simulink model "pumacherif"  (R2023b)
settings: Solver=VariableStepAuto  StartTime=0.0  StopTime=10.0  RelTol=1e-3  AbsTol=1e-3  EnableMultiTasking=on
undefined symbols (not defined in the file): X, Y, Z
libraries: sm_lib x29, nesl_utility x10
settings Model: Creator=echerif913  LastModifiedBy=enzoc
settings SolverCC: AutoScaleAbsTol=off  AlgebraicLoopSolver=TrustRegion  MaxZcPerStep=1
settings DataIOCC: LimitDataPoints=on  MaxDataPoints=10000
settings OptimizationCC: ReuseModelBlockBuffer=off  LifeSpan=inf
settings DebuggingCC: UnconnectedInputMsg=warning  UnconnectedOutputMsg=warning  UnconnectedLineMsg=warning  AllowSymbolicDim=off  SFUnexpectedBacktrackingDiag=warning  SFNoUnconditionalDefaultTransitionDiag=warning  SFExecutionAtInitializationDiag=none  ArithmeticOperatorsInVariantConditions=warning
settings ModelReferenceCC: EnableRefExpFcnMdlSchedulingChecks=on
settings SFSimCC: SimUseLocalCustomCode=off  CustomCodeUndefinedFunction=UseInterfaceOnly
settings RTWCC: RTWUseLocalCustomCode=off  DLArmComputeVersion=19.05
settings CodeAppCC: StateflowObjectComments=on
settings GRTTargetCC: TargetLangStandard=C89/C90 (ANSI)
settings ConfigComp: CovMetricSettings=dw  CovSaveCumulativeToWorkspaceVar=on  CovSaveSingleToWorkspaceVar=on  CovExternalEMLEnable=off  CovSFcnEnable=off
settings SimscapeCC: SimscapeLogType=all  SimscapeLogSimulationStatistics=on  SimscapeLogDataHistory=10000

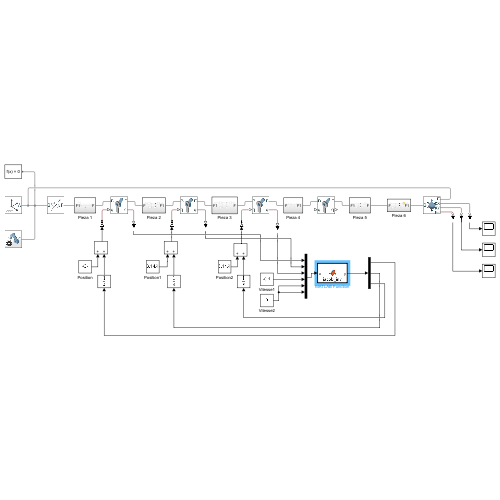
[thumbnail: Simulink's stored preview of the top-level diagram]
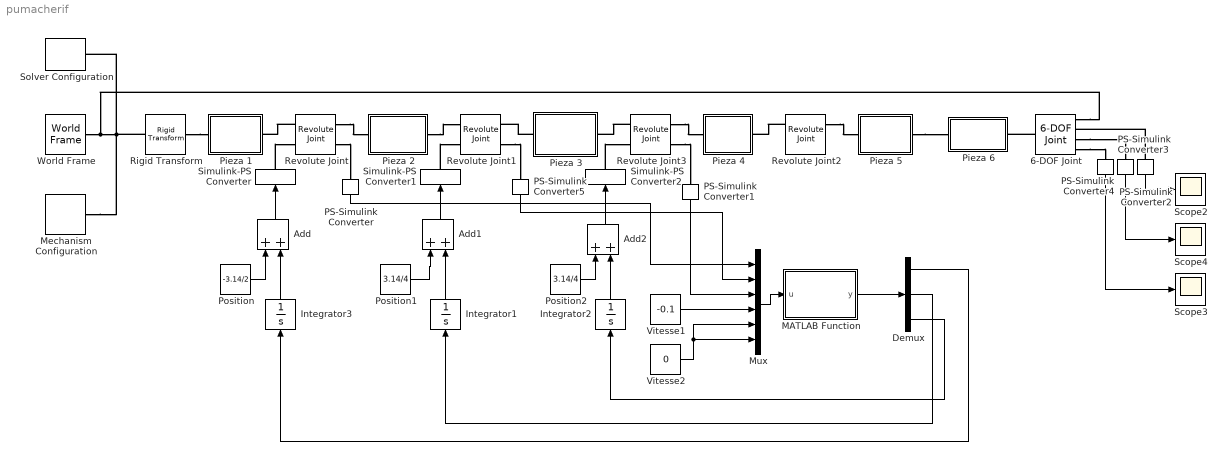
== system pumacherif ==
  6-DOF Joint : sm_lib/Joints/6-DOF Joint  JointMode=Normal  SenseConstraintForce=off  SenseConstraintForceX=off  SenseConstraintForceY=off  SenseConstraintForceZ=off  SenseConstraintTorque=off  SenseConstraintTorqueX=off  SenseConstraintTorqueY=off  SenseConstraintTorqueZ=off  SenseTotalForce=off  SenseTotalForceX=off  SenseTotalForceY=off  SenseTotalForceZ=off  SenseTotalTorque=off  SenseTotalTorqueX=off  SenseTotalTorqueY=off  SenseTotalTorqueZ=off  CompositeWrenchDir=FollowerOnBase  CompositeWrenchFrame=BaseFrame  PxEquilibriumPosition=0  PxEquilibriumPositionUnits=m  PxSpringStiffness=0  PxSpringStiffnessUnits=N/m  PxDampingCoefficient=0  PxDampingCoefficientUnits=N/(m/s)  PxTorqueActuationMode=NoTorque  PxMotionActuationMode=ComputedMotion  PxSensePosition=on  PxSenseVelocity=off  PxSenseAcceleration=off  PxSenseTorqueForce=off  PxSenseLowerLimitTorqueForce=off  PxSenseUpperLimitTorqueForce=off  PxLowerLimitSpecify=off  PxLowerLimitBound=-1  PxLowerLimitBoundUnits=m  PxLowerLimitStiffness=1e6  PxLowerLimitStiffnessUnits=N/m  PxLowerLimitDamping=1e3  PxLowerLimitDampingUnits=N/(m/s)  PxLowerLimitTransitionRegionWidth=1e-4  PxLowerLimitTransitionRegionWidthUnits=m  PxUpperLimitSpecify=off  PxUpperLimitBound=1  PxUpperLimitBoundUnits=m  PxUpperLimitStiffness=1e6  PxUpperLimitStiffnessUnits=N/m  PxUpperLimitDamping=1e3  PxUpperLimitDampingUnits=N/(m/s)  PxUpperLimitTransitionRegionWidth=1e-4  PxUpperLimitTransitionRegionWidthUnits=m  PxPositionTargetSpecify=off  PxPositionTargetPriority=High  PxPositionTargetValue=0  PxPositionTargetValueUnits=m  PxVelocityTargetSpecify=off  PxVelocityTargetPriority=High  PxVelocityTargetValue=0  PxVelocityTargetValueUnits=m/s  PyEquilibriumPosition=0  PyEquilibriumPositionUnits=m  PySpringStiffness=0  PySpringStiffnessUnits=N/m  PyDampingCoefficient=0  PyDampingCoefficientUnits=N/(m/s)  PyTorqueActuationMode=NoTorque  PyMotionActuationMode=ComputedMotion  PySensePosition=on  PySenseVelocity=off  PySenseAcceleration=off  PySenseTorqueForce=off  PySenseLowerLimitTorqueForce=off  PySenseUpperLimitTorqueForce=off  PyLowerLimitSpecify=off  PyLowerLimitBound=-1  PyLowerLimitBoundUnits=m  PyLowerLimitStiffness=1e6  PyLowerLimitStiffnessUnits=N/m  PyLowerLimitDamping=1e3  PyLowerLimitDampingUnits=N/(m/s)  PyLowerLimitTransitionRegionWidth=1e-4  PyLowerLimitTransitionRegionWidthUnits=m  PyUpperLimitSpecify=off  PyUpperLimitBound=1  PyUpperLimitBoundUnits=m  PyUpperLimitStiffness=1e6  PyUpperLimitStiffnessUnits=N/m  PyUpperLimitDamping=1e3  PyUpperLimitDampingUnits=N/(m/s)  PyUpperLimitTransitionRegionWidth=1e-4  PyUpperLimitTransitionRegionWidthUnits=m  PyPositionTargetSpecify=off  PyPositionTargetPriority=High  PyPositionTargetValue=0  PyPositionTargetValueUnits=m  PyVelocityTargetSpecify=off  PyVelocityTargetPriority=High  PyVelocityTargetValue=0  PyVelocityTargetValueUnits=m/s  PzEquilibriumPosition=0  PzEquilibriumPositionUnits=m  PzSpringStiffness=0  PzSpringStiffnessUnits=N/m  PzDampingCoefficient=0  PzDampingCoefficientUnits=N/(m/s)  PzTorqueActuationMode=NoTorque  PzMotionActuationMode=ComputedMotion  PzSensePosition=on  PzSenseVelocity=off  PzSenseAcceleration=off  PzSenseTorqueForce=off  PzSenseLowerLimitTorqueForce=off  PzSenseUpperLimitTorqueForce=off  PzLowerLimitSpecify=off  PzLowerLimitBound=-1  PzLowerLimitBoundUnits=m  PzLowerLimitStiffness=1e6  PzLowerLimitStiffnessUnits=N/m  PzLowerLimitDamping=1e3  PzLowerLimitDampingUnits=N/(m/s)  PzLowerLimitTransitionRegionWidth=1e-4  PzLowerLimitTransitionRegionWidthUnits=m  PzUpperLimitSpecify=off  PzUpperLimitBound=1  PzUpperLimitBoundUnits=m  PzUpperLimitStiffness=1e6  PzUpperLimitStiffnessUnits=N/m  PzUpperLimitDamping=1e3  PzUpperLimitDampingUnits=N/(m/s)  PzUpperLimitTransitionRegionWidth=1e-4  PzUpperLimitTransitionRegionWidthUnits=m  PzPositionTargetSpecify=off  PzPositionTargetPriority=High  PzPositionTargetValue=0  PzPositionTargetValueUnits=m  PzVelocityTargetSpecify=off  PzVelocityTargetPriority=High  PzVelocityTargetValue=0  PzVelocityTargetValueUnits=m/s  SphEqPosRotationMethod=None  SphEqPosRotationAngleUnits=deg  SphEqPosRotationStandardAxis=+Z  SphEqPosRotationAngle=0.0  SphEqPosRotationArbitraryAxis=[0 0 1]  SphEqPosFollAlignAxisA=+X  SphEqPosBaseAlignAxisA=+Y  SphEqPosFollAlignAxisB=+Y  SphEqPosBaseAlignAxisB=+Z  SphEqPosRotationSequenceAxes=FollowerAxes  SphEqPosRotationSequence=XYX  SphEqPosRotationSequenceAngles=[0 0 0]  SphEqPosRotationSequenceAnglesUnits=deg  SphEqPosRotationMatrix=[1 0 0; 0 1 0; 0 0 1]  SphEqPosQuaternion=[1 0 0 0]  SphSpringStiffness=0  SphSpringStiffnessUnits=N*m/deg  SphDampingCoefficient=0  SphDampingCoefficientUnits=N*m/(deg/s)  SphActuateTorqueX=off  SphActuateTorqueY=off  SphActuateTorqueZ=off  SphActuateTorque=off  SphTorqueActuationMode=NoTorque  SphMotionActuationMode=ComputedMotion  SphActuationFrame=BaseFrame  SphSensePosition=off  SphSenseVelocityX=off  SphSenseVelocityY=off  SphSenseVelocityZ=off  SphSenseVelocity=off  SphSenseAccelerationX=off  SphSenseAccelerationY=off  SphSenseAccelerationZ=off  SphSenseAcceleration=off  SphSenseTorqueX=off  SphSenseTorqueY=off  SphSenseTorqueZ=off  SphSenseTorqueForce=off  SphSenseLowerLimitTorqueMag=off  SphSenseUpperLimitTorqueMag=off  SphSensingFrame=BaseFrame  SphLowerLimitSpecify=off  SphLowerLimitBound=15  SphLowerLimitBoundUnits=deg  SphLowerLimitStiffness=1e4  SphLowerLimitStiffnessUnits=N*m/deg  SphLowerLimitDamping=10  SphLowerLimitDampingUnits=N*m/(deg/s)  SphLowerLimitTransitionRegionWidth=0.1  SphLowerLimitTransitionRegionWidthUnits=deg  SphUpperLimitSpecify=off  SphUpperLimitBound=45  SphUpperLimitBoundUnits=deg  SphUpperLimitStiffness=1e4  SphUpperLimitStiffnessUnits=N*m/deg  SphUpperLimitDamping=10  SphUpperLimitDampingUnits=N*m/(deg/s)  SphUpperLimitTransitionRegionWidth=0.1  SphUpperLimitTransitionRegionWidthUnits=deg  SphPositionTargetRotationMethod=None  SphPositionTargetRotationAngleUnits=deg  SphPositionTargetRotationStandardAxis=+Z  SphPositionTargetRotationAngle=0.0  SphPositionTargetRotationArbitraryAxis=[0 0 1]  SphPositionTargetFollAlignAxisA=+X  SphPositionTargetBaseAlignAxisA=+Y  SphPositionTargetFollAlignAxisB=+Y  SphPositionTargetBaseAlignAxisB=+Z  SphPositionTargetRotationSequenceAxes=FollowerAxes  SphPositionTargetRotationSequence=XYX  SphPositionTargetRotationSequenceAngles=[0 0 0]  SphPositionTargetRotationSequenceAnglesUnits=deg  SphPositionTargetRotationMatrix=[1 0 0; 0 1 0; 0 0 1]  SphPositionTargetQuaternion=[1 0 0 0]  SphPositionTargetSpecify=off  SphPositionTargetPriority=High  SphVelocityTargetValue=[0 0 0]  SphVelocityTargetValueUnits=deg/s  SphVelocityTargetSpecify=off  SphVelocityTargetPriority=High  SphVelocityTargetInFollowerFrame=on
  Add : Sum
  Add1 : Sum
  Add2 : Sum
  Demux : Demux  Outputs=3
  Integrator1 : Integrator
  Integrator2 : Integrator
  Integrator3 : Integrator
  MATLAB Function : MATLAB Function  TreatAsAtomicUnit=on
  Mechanism Configuration : sm_lib/Utilities/Mechanism Configuration  UniformGravity=Constant  GravityVector=[0 0 -9.80665]  GravityVectorUnits=m/s^2  LinearizationDelta=0.001  JointModeTransitionNonlinearIterations=2
  Mux : Mux  Inputs=6
  PS-Simulink Converter{,1..5} (6 alike) : nesl_utility/PS-Simulink Converter  PhysicalDomain=network_engine_domain  SubClassName=ps_output  LeftPortType=input  RightPortType=output  PseudoPeriodic=off  Frequencies=[]  VectorFormat=inherit  Unit=inherit  AffineConversion=off
  Pieza 1 : Subsystem
  Pieza 2 : Subsystem
  Pieza 3 : Subsystem
  Pieza 4 : Subsystem
  Pieza 5 : Subsystem
  Pieza 6 : Subsystem
  Position : Constant  Value=-3.14/2
  Position1 : Constant  Value=3.14/4
  Position2 : Constant  Value=3.14/4
  Revolute Joint{,1..3} (4 alike) : sm_lib/Joints/Revolute Joint  JointMode=Normal  SenseConstraintForce=off  SenseConstraintForceX=off  SenseConstraintForceY=off  SenseConstraintForceZ=off  SenseConstraintTorque=off  SenseConstraintTorqueX=off  SenseConstraintTorqueY=off  SenseConstraintTorqueZ=off  SenseTotalForce=off  SenseTotalForceX=off  SenseTotalForceY=off  SenseTotalForceZ=off  SenseTotalTorque=off  SenseTotalTorqueX=off  SenseTotalTorqueY=off  SenseTotalTorqueZ=off  CompositeWrenchDir=FollowerOnBase  CompositeWrenchFrame=BaseFrame  EquilibriumPosition=0  EquilibriumPositionUnits=deg  SpringStiffness=0  SpringStiffnessUnits=N*m/deg  DampingCoefficient=0  DampingCoefficientUnits=N*m/(deg/s)  TorqueActuationMode=ComputedTorque  MotionActuationMode=InputMotion  SensePosition=on  SenseVelocity=off  SenseAcceleration=off  SenseTorqueForce=off  SenseLowerLimitTorqueForce=off  SenseUpperLimitTorqueForce=off  LowerLimitSpecify=off  LowerLimitBound=-90  LowerLimitBoundUnits=deg  LowerLimitStiffness=1e4  LowerLimitStiffnessUnits=N*m/deg  LowerLimitDamping=10  LowerLimitDampingUnits=N*m/(deg/s)  LowerLimitTransitionRegionWidth=0.1  LowerLimitTransitionRegionWidthUnits=deg  UpperLimitSpecify=off  UpperLimitBound=90  UpperLimitBoundUnits=deg  UpperLimitStiffness=1e4  UpperLimitStiffnessUnits=N*m/deg  UpperLimitDamping=10  UpperLimitDampingUnits=N*m/(deg/s)  UpperLimitTransitionRegionWidth=0.1  UpperLimitTransitionRegionWidthUnits=deg  PositionTargetSpecify=off  PositionTargetPriority=High  PositionTargetValue=0  PositionTargetValueUnits=deg  VelocityTargetSpecify=off  VelocityTargetPriority=High  VelocityTargetValue=0  VelocityTargetValueUnits=deg/s
  Rigid Transform : sm_lib/Frames and Transforms/Rigid Transform  TranslationMethod=None  TranslationStandardOffset=0  TranslationStandardOffsetUnits=m  TranslationStandardAxis=+Z  TranslationCartesianOffset=[0 0 0]  TranslationCartesianOffsetUnits=m  TranslationROffset=0  TranslationROffsetUnits=m  TranslationZOffset=0  TranslationZOffsetUnits=m  TranslationThetaOffset=0  TranslationThetaOffsetUnits=deg  RotationMethod=RotationMatrix  RotationAngleUnits=deg  RotationStandardAxis=+Z  RotationAngle=0.0  RotationArbitraryAxis=[0 0 1]  FollAlignAxisA=+X  BaseAlignAxisA=+Y  FollAlignAxisB=+Y  BaseAlignAxisB=+Z  RotationSequenceAxes=FollowerAxes  RotationSequence=XYX  RotationSequenceAngles=[0 0 0]  RotationSequenceAnglesUnits=deg  RotationMatrix=[0 0 1; 1 0 0; 0 1 0]  Quaternion=[1 0 0 0]
  Scope2 : Scope
  Scope3 : Scope
  Scope4 : Scope
  Simulink-PS Converter : nesl_utility/Simulink-PS Converter  PhysicalDomain=network_engine_domain  SubClassName=ps_input  LeftPortType=input  RightPortType=output  PseudoPeriodic=off  Frequencies=[]  NoiseDistribution=none  NoiseParameters=[]  Unit=rad  AffineConversion=off  FilteringAndDerivatives=filter  SimscapeFilterOrder=2  InputFilterTimeConstant=0.001  UdotUserProvided=2
  Simulink-PS Converter1 : nesl_utility/Simulink-PS Converter  PhysicalDomain=network_engine_domain  SubClassName=ps_input  LeftPortType=input  RightPortType=output  PseudoPeriodic=off  Frequencies=[]  NoiseDistribution=none  NoiseParameters=[]  Unit=rad  AffineConversion=off  FilteringAndDerivatives=filter  SimscapeFilterOrder=2  InputFilterTimeConstant=0.001  UdotUserProvided=0
  Simulink-PS Converter2 : nesl_utility/Simulink-PS Converter  PhysicalDomain=network_engine_domain  SubClassName=ps_input  LeftPortType=input  RightPortType=output  PseudoPeriodic=off  Frequencies=[]  NoiseDistribution=none  NoiseParameters=[]  Unit=rad  AffineConversion=off  FilteringAndDerivatives=filter  SimscapeFilterOrder=2  InputFilterTimeConstant=0.001  UdotUserProvided=0
  Solver Configuration : nesl_utility/Solver Configuration  PhysicalDomain=network_engine_domain  SubClassName=solver  LeftPortType=input  RightPortType=generic  Tones=[]  Harmonics=[]  SimulateNoise=off  Profile=off  UseLocalSampling=off  EnableSwitchedLinearOptims=on  FrequencyDomain=off  UseCCode=off  RelTol=0.001  AbsTol=1e-06  MinStep=1e-09  ToWorkspace=off  RevertToSquareIcSolve=off  NumHomotopyIterations=100  PhasorMode=off  PhasorModeNumHarmonics=1  ConsistencySolver=NEWTON_XTOL_AFTER_FTOL  IndexReductionMethod=DerivativeReplacement  DoDC=off  ResidualTolerance=1e-09  ConsistencyTolSource=GLOBAL  ConsistencyAbsTol=0.001  ConsistencyRelTol=0.001  ConsistencyTolFactor=0.001  UseLocalSolver=off  LocalSolverChoice=NE_BACKWARD_EULER_ADVANCER  ResolveIndetEquations=on  FunctionEvalNumThread=1  LocalSolverSampleTime=0.001  DoFixedCost=off  MaxNonlinIter=3  MaxModeIter=2  ComputeImpulses=off  ImpulseIterations=2  LinearAlgebra=Sparse  LinearAlgebraNumThread=0  EquationFormulation=NE_TIME_EF  DelaysMemoryBudget=1024  AutomaticFiltering=on  FilteringTimeConstant=0.001  PartitionStorageMethod=AS_NEEDED  PartitionMemoryBudget=1024  PartitionMethod=FAST  MultibodyUseLocalSolver=off  MultibodyLocalSolverChoice=ODE1  MultibodyLocalSolverSampleTime=0.001
  Vitesse1 : Constant  Value=-0.1
  Vitesse2 : Constant  Value=0
  World Frame : sm_lib/Frames and Transforms/World Frame
  wires:
  Add/1 -> Simulink-PS Converter/1
  Position/1 -> Add/1
  Integrator3/1 -> Add/2
  PS-Simulink Converter2/1 -> Scope2/1
  PS-Simulink Converter3/1 -> Scope4/1
  PS-Simulink Converter4/1 -> Scope3/1
  Integrator1/1 -> Add1/2
  Add1/1 -> Simulink-PS Converter1/1
  Position1/1 -> Add1/1
  Integrator2/1 -> Add2/2
  Add2/1 -> Simulink-PS Converter2/1
  Position2/1 -> Add2/1
  Mux/1 -> MATLAB Function/1(u)
  MATLAB Function/1(y) -> Demux/1
  PS-Simulink Converter/1 -> Mux/1
  PS-Simulink Converter5/1 -> Mux/2
  PS-Simulink Converter1/1 -> Mux/3
  Vitesse1/1 -> Mux/4
  Vitesse2/1 -> Mux/5, Mux/6
  Demux/1 -> Integrator3/1
  Demux/2 -> Integrator1/1
  Demux/3 -> Integrator2/1
  connections:
  World Frame/RConn1 -- 6-DOF Joint/RConn1 -- Mechanism Configuration/RConn1 -- Rigid Transform/LConn1 -- Solver Configuration/RConn1
  Rigid Transform/RConn1 -- Pieza 1/LConn1
  Revolute Joint/LConn1 -- Pieza 1/RConn1
  Revolute Joint/RConn1 -- Pieza 2/LConn1
  Pieza 2/RConn1 -- Revolute Joint1/LConn1
  Revolute Joint3/LConn1 -- Pieza 3/RConn1
  Revolute Joint3/RConn1 -- Pieza 4/LConn1
  Pieza 3/LConn1 -- Revolute Joint1/RConn1
  Revolute Joint2/RConn1 -- Pieza 5/LConn1
  Revolute Joint2/LConn1 -- Pieza 4/RConn1
  Pieza 5/RConn1 -- Pieza 6/LConn1
  Revolute Joint/RConn2 -- PS-Simulink Converter/LConn1
  Simulink-PS Converter/RConn1 -- Revolute Joint/LConn2
  6-DOF Joint/LConn1 -- Pieza 6/RConn1
  PS-Simulink Converter2/LConn1 -- 6-DOF Joint/RConn2
  6-DOF Joint/RConn4 -- PS-Simulink Converter4/LConn1
  6-DOF Joint/RConn3 -- PS-Simulink Converter3/LConn1
  Simulink-PS Converter1/RConn1 -- Revolute Joint1/LConn2
  Simulink-PS Converter2/RConn1 -- Revolute Joint3/LConn2
  Revolute Joint1/RConn2 -- PS-Simulink Converter5/LConn1
  Revolute Joint3/RConn2 -- PS-Simulink Converter1/LConn1

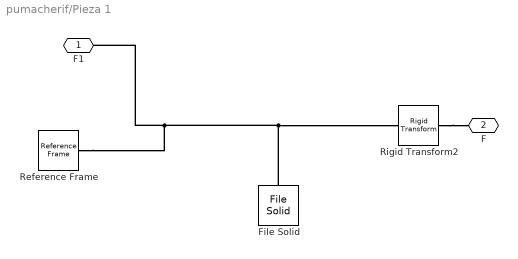
== system pumacherif/Pieza 1 ==
  File Solid : sm_lib/Body Elements/File Solid  ExtGeomFileName=C:\Users\enzoc\Desktop\TP PUMA\puma\Pieza 1_Predeterminado_sldprt.STL  UnitType=Custom  ExtGeomFileUnits=in  StepReaderType=HEX  ExportConvexHullGeometry=off  InertiaType=Custom  Mass=1  MassUnits=kg  CenterOfMass=[0 0 0]  CenterOfMassUnits=m  MomentsOfInertia=[1 1 1]  MomentsOfInertiaUnits=kg*m^2  ProductsOfInertia=[0 0 0]  ProductsOfInertiaUnits=kg*m^2  BasedOnType=DensityFromFile  Density=1000  DensityUnits=kg/m^3  DoExposeReferenceFrame=on  SerializedFrames=<Frames><Frame><Id>Frame1</Id><Value><Name>F1</Name><Origin><Source>ReferenceFrame</Source><FeatureName></FeatureName></Origin><PrimaryAxis><DefinedDirection>-Y</DefinedDirection><Source>ReferenceFrame</Source><SourceDirection>+Z</SourceDirection><FeatureName></FeatureName></PrimaryAxis><SecondaryAxis><DefinedDirection>+X</DefinedDirection><Source>ReferenceFrame</Source><SourceDirection>+X</SourceDirection><FeatureName></FeatureName></SecondaryAxis></Value></Frame></Frames>  GraphicType=FromGeometry  MarkerShape=Sphere  MarkerSize=10  GraphicVisPropType=SimpleVisualProperties  GraphicDiffuseColor=[1.0 0.0 1.0]  GraphicSpecularColor=[0.5 0.5 0.5 1.0]  GraphicAmbientColor=[0.15 0.15 0.15 1.0]  GraphicEmissiveColor=[0.0 0.0 0.0 1.0]  GraphicShininess=75  GraphicOpacity=1.0
  Reference Frame : sm_lib/Frames and Transforms/Reference Frame
  Rigid Transform2 : sm_lib/Frames and Transforms/Rigid Transform  TranslationMethod=None  TranslationStandardOffset=24  TranslationStandardOffsetUnits=m  TranslationStandardAxis=+Y  TranslationCartesianOffset=[0 0.624 0]  TranslationCartesianOffsetUnits=m  TranslationROffset=0  TranslationROffsetUnits=m  TranslationZOffset=0  TranslationZOffsetUnits=m  TranslationThetaOffset=0  TranslationThetaOffsetUnits=deg  RotationMethod=RotationMatrix  RotationAngleUnits=deg  RotationStandardAxis=+Z  RotationAngle=0.0  RotationArbitraryAxis=[0 0 1]  FollAlignAxisA=+Z  BaseAlignAxisA=+Y  FollAlignAxisB=+Y  BaseAlignAxisB=+Z  RotationSequenceAxes=FollowerAxes  RotationSequence=XYX  RotationSequenceAngles=[0 0 0]  RotationSequenceAnglesUnits=deg  RotationMatrix=[0 -1 0; 0 0 1; -1 0 0]  Quaternion=[1 0 0 0]
  F1 : PMIOPort  Side=Left
  F : PMIOPort  Port=2  Side=Right
  connections:
  Rigid Transform2/RConn1 -- F/RConn1
  File Solid/RConn1 -- Reference Frame/RConn1 -- F1/RConn1 -- Rigid Transform2/LConn1

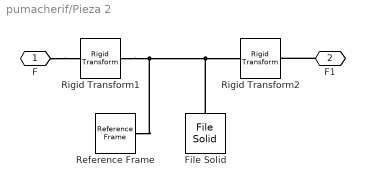
== system pumacherif/Pieza 2 ==
  File Solid : sm_lib/Body Elements/File Solid  ExtGeomFileName=C:\Users\enzoc\Desktop\TP PUMA\puma\Pieza 2_Predeterminado_sldprt.STL  UnitType=Custom  ExtGeomFileUnits=in  StepReaderType=HEX  ExportConvexHullGeometry=off  InertiaType=Custom  Mass=1  MassUnits=kg  CenterOfMass=[0 0 0]  CenterOfMassUnits=m  MomentsOfInertia=[1 1 1]  MomentsOfInertiaUnits=kg*m^2  ProductsOfInertia=[0 0 0]  ProductsOfInertiaUnits=kg*m^2  BasedOnType=DensityFromFile  Density=1000  DensityUnits=kg/m^3  DoExposeReferenceFrame=on  SerializedFrames=<Frames/>  GraphicType=FromGeometry  MarkerShape=Sphere  MarkerSize=10  GraphicVisPropType=SimpleVisualProperties  GraphicDiffuseColor=[0.4 1.0 0.0]  GraphicSpecularColor=[0.5 0.5 0.5 1.0]  GraphicAmbientColor=[0.15 0.15 0.15 1.0]  GraphicEmissiveColor=[0.0 0.0 0.0 1.0]  GraphicShininess=75  GraphicOpacity=1.0
  Reference Frame : sm_lib/Frames and Transforms/Reference Frame
  Rigid Transform1 : sm_lib/Frames and Transforms/Rigid Transform  TranslationMethod=StandardAxis  TranslationStandardOffset=0.624  TranslationStandardOffsetUnits=m  TranslationStandardAxis=+Z  TranslationCartesianOffset=[0 0 0]  TranslationCartesianOffsetUnits=m  TranslationROffset=0  TranslationROffsetUnits=m  TranslationZOffset=0  TranslationZOffsetUnits=m  TranslationThetaOffset=0  TranslationThetaOffsetUnits=deg  RotationMethod=RotationMatrix  RotationAngleUnits=deg  RotationStandardAxis=+Z  RotationAngle=0.0  RotationArbitraryAxis=[0 0 1]  FollAlignAxisA=+X  BaseAlignAxisA=+Y  FollAlignAxisB=+Y  BaseAlignAxisB=+Z  RotationSequenceAxes=FollowerAxes  RotationSequence=XYX  RotationSequenceAngles=[0 0 0]  RotationSequenceAnglesUnits=deg  RotationMatrix=[-1 0 0; 0 0 -1; 0 -1 0]  Quaternion=[1 0 0 0]
  Rigid Transform2 : sm_lib/Frames and Transforms/Rigid Transform  TranslationMethod=None  TranslationStandardOffset=0.142  TranslationStandardOffsetUnits=m  TranslationStandardAxis=+Z  TranslationCartesianOffset=[0 0 0]  TranslationCartesianOffsetUnits=m  TranslationROffset=0  TranslationROffsetUnits=m  TranslationZOffset=0  TranslationZOffsetUnits=m  TranslationThetaOffset=0  TranslationThetaOffsetUnits=deg  RotationMethod=RotationMatrix  RotationAngleUnits=deg  RotationStandardAxis=+Z  RotationAngle=0.0  RotationArbitraryAxis=[0 0 1]  FollAlignAxisA=+X  BaseAlignAxisA=+Y  FollAlignAxisB=+Y  BaseAlignAxisB=+Z  RotationSequenceAxes=FollowerAxes  RotationSequence=XYX  RotationSequenceAngles=[0 0 0]  RotationSequenceAnglesUnits=deg  RotationMatrix="[0 0 -1; 0  1 0; 1 0 0]"  Quaternion=[1 0 0 0]
  F : PMIOPort  Side=Left
  F1 : PMIOPort  Port=2  Side=Right
  connections:
  F1/RConn1 -- Rigid Transform2/RConn1
  F/RConn1 -- Rigid Transform1/LConn1
  Rigid Transform1/RConn1 -- Reference Frame/RConn1 -- File Solid/RConn1 -- Rigid Transform2/LConn1

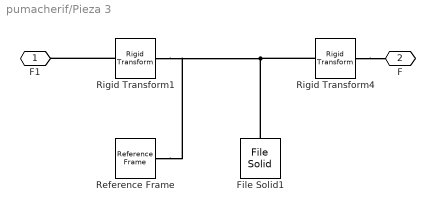
== system pumacherif/Pieza 3 ==
  File Solid1 : sm_lib/Body Elements/File Solid  ExtGeomFileName=C:\Users\enzoc\Desktop\TP PUMA\puma\Pieza 3_Predeterminado_sldprt.STL  UnitType=Custom  ExtGeomFileUnits=in  StepReaderType=HEX  ExportConvexHullGeometry=off  InertiaType=Custom  Mass=1  MassUnits=kg  CenterOfMass=[0 0 0]  CenterOfMassUnits=m  MomentsOfInertia=[1 1 1]  MomentsOfInertiaUnits=kg*m^2  ProductsOfInertia=[0 0 0]  ProductsOfInertiaUnits=kg*m^2  BasedOnType=DensityFromFile  Density=1000  DensityUnits=kg/m^3  DoExposeReferenceFrame=on  SerializedFrames=<Frames/>  GraphicType=FromGeometry  MarkerShape=Sphere  MarkerSize=10  GraphicVisPropType=SimpleVisualProperties  GraphicDiffuseColor=[0.0 0.0 1.0]  GraphicSpecularColor=[0.5 0.5 0.5 1.0]  GraphicAmbientColor=[0.15 0.15 0.15 1.0]  GraphicEmissiveColor=[0.0 0.0 0.0 1.0]  GraphicShininess=75  GraphicOpacity=1.0
  Reference Frame : sm_lib/Frames and Transforms/Reference Frame
  Rigid Transform1 : sm_lib/Frames and Transforms/Rigid Transform  TranslationMethod=StandardAxis  TranslationStandardOffset=0.142  TranslationStandardOffsetUnits=m  TranslationStandardAxis=+Z  TranslationCartesianOffset=[0 0 0]  TranslationCartesianOffsetUnits=m  TranslationROffset=0  TranslationROffsetUnits=m  TranslationZOffset=0  TranslationZOffsetUnits=m  TranslationThetaOffset=0  TranslationThetaOffsetUnits=deg  RotationMethod=RotationMatrix  RotationAngleUnits=deg  RotationStandardAxis=+Z  RotationAngle=0.0  RotationArbitraryAxis=[0 0 1]  FollAlignAxisA=+X  BaseAlignAxisA=+Y  FollAlignAxisB=+Y  BaseAlignAxisB=+Z  RotationSequenceAxes=FollowerAxes  RotationSequence=XYX  RotationSequenceAngles=[0 0 0]  RotationSequenceAnglesUnits=deg  RotationMatrix=[0 0 1; 0 1 0; -1 0 0]  Quaternion=[1 0 0 0]
  Rigid Transform4 : sm_lib/Frames and Transforms/Rigid Transform  TranslationMethod=StandardAxis  TranslationStandardOffset=0.432  TranslationStandardOffsetUnits=m  TranslationStandardAxis=+Z  TranslationCartesianOffset=[0 0 0]  TranslationCartesianOffsetUnits=m  TranslationROffset=0  TranslationROffsetUnits=m  TranslationZOffset=0  TranslationZOffsetUnits=m  TranslationThetaOffset=0  TranslationThetaOffsetUnits=deg  RotationMethod=RotationMatrix  RotationAngleUnits=deg  RotationStandardAxis=+Z  RotationAngle=0.0  RotationArbitraryAxis=[0 0 1]  FollAlignAxisA=+X  BaseAlignAxisA=+Y  FollAlignAxisB=+Y  BaseAlignAxisB=+Z  RotationSequenceAxes=FollowerAxes  RotationSequence=XYX  RotationSequenceAngles=[0 0 0]  RotationSequenceAnglesUnits=deg  RotationMatrix=[0 0 1; -1 0 0; 0 -1 0]  Quaternion=[1 0 0 0]
  F1 : PMIOPort  Side=Left
  F : PMIOPort  Port=2  Side=Right
  connections:
  Rigid Transform4/LConn1 -- Rigid Transform1/RConn1 -- Reference Frame/RConn1 -- File Solid1/RConn1
  Rigid Transform4/RConn1 -- F/RConn1
  Rigid Transform1/LConn1 -- F1/RConn1

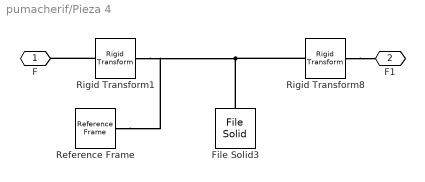
== system pumacherif/Pieza 4 ==
  File Solid3 : sm_lib/Body Elements/File Solid  ExtGeomFileName=C:\Users\enzoc\Desktop\TP PUMA\puma\Pieza 4_Predeterminado_sldprt.STL  UnitType=Custom  ExtGeomFileUnits=in  StepReaderType=HEX  ExportConvexHullGeometry=off  InertiaType=Custom  Mass=1  MassUnits=kg  CenterOfMass=[0 0 0]  CenterOfMassUnits=m  MomentsOfInertia=[1 1 1]  MomentsOfInertiaUnits=kg*m^2  ProductsOfInertia=[0 0 0]  ProductsOfInertiaUnits=kg*m^2  BasedOnType=DensityFromFile  Density=1000  DensityUnits=kg/m^3  DoExposeReferenceFrame=on  SerializedFrames=<Frames/>  GraphicType=FromGeometry  MarkerShape=Sphere  MarkerSize=10  GraphicVisPropType=SimpleVisualProperties  GraphicDiffuseColor=[0.5 0.5 0.5]  GraphicSpecularColor=[0.5 0.5 0.5 1.0]  GraphicAmbientColor=[0.15 0.15 0.15 1.0]  GraphicEmissiveColor=[0.0 0.0 0.0 1.0]  GraphicShininess=75  GraphicOpacity=1.0
  Reference Frame : sm_lib/Frames and Transforms/Reference Frame
  Rigid Transform1 : sm_lib/Frames and Transforms/Rigid Transform  TranslationMethod=None  TranslationStandardOffset=0  TranslationStandardOffsetUnits=m  TranslationStandardAxis=+Z  TranslationCartesianOffset=[0 0 0]  TranslationCartesianOffsetUnits=m  TranslationROffset=0  TranslationROffsetUnits=m  TranslationZOffset=0  TranslationZOffsetUnits=m  TranslationThetaOffset=0  TranslationThetaOffsetUnits=deg  RotationMethod=RotationMatrix  RotationAngleUnits=deg  RotationStandardAxis=+Z  RotationAngle=0.0  RotationArbitraryAxis=[0 0 1]  FollAlignAxisA=+X  BaseAlignAxisA=+Y  FollAlignAxisB=+Y  BaseAlignAxisB=+Z  RotationSequenceAxes=FollowerAxes  RotationSequence=XYX  RotationSequenceAngles=[0 0 0]  RotationSequenceAnglesUnits=deg  RotationMatrix=[0 -1 0; 0 0 -1; 1 0 0]  Quaternion=[1 0 0 0]
  Rigid Transform8 : sm_lib/Frames and Transforms/Rigid Transform  TranslationMethod=Cartesian  TranslationStandardOffset=0  TranslationStandardOffsetUnits=m  TranslationStandardAxis=+Z  TranslationCartesianOffset=[0.038 -0.352 0]  TranslationCartesianOffsetUnits=m  TranslationROffset=0  TranslationROffsetUnits=m  TranslationZOffset=0  TranslationZOffsetUnits=m  TranslationThetaOffset=0  TranslationThetaOffsetUnits=deg  RotationMethod=None  RotationAngleUnits=deg  RotationStandardAxis=+Z  RotationAngle=0.0  RotationArbitraryAxis=[0 0 1]  FollAlignAxisA=+X  BaseAlignAxisA=+Y  FollAlignAxisB=+Y  BaseAlignAxisB=+Z  RotationSequenceAxes=FollowerAxes  RotationSequence=XYX  RotationSequenceAngles=[0 0 0]  RotationSequenceAnglesUnits=deg  RotationMatrix="[0 0 1 ; 1 0  0;0 1 0]"  Quaternion=[1 0 0 0]
  F : PMIOPort  Side=Left
  F1 : PMIOPort  Port=2  Side=Right
  connections:
  Rigid Transform8/LConn1 -- Rigid Transform1/RConn1 -- Reference Frame/RConn1 -- File Solid3/RConn1
  Rigid Transform8/RConn1 -- F1/RConn1
  Rigid Transform1/LConn1 -- F/RConn1

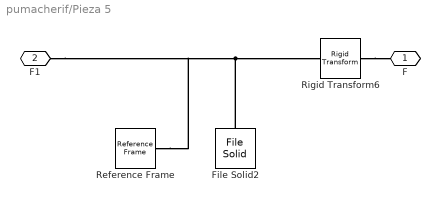
== system pumacherif/Pieza 5 ==
  File Solid2 : sm_lib/Body Elements/File Solid  ExtGeomFileName=C:\Users\enzoc\Desktop\TP PUMA\puma\Pieza 5_Predeterminado_sldprt.STL  UnitType=Custom  ExtGeomFileUnits=in  StepReaderType=HEX  ExportConvexHullGeometry=off  InertiaType=Custom  Mass=1  MassUnits=kg  CenterOfMass=[0 0 0]  CenterOfMassUnits=m  MomentsOfInertia=[1 1 1]  MomentsOfInertiaUnits=kg*m^2  ProductsOfInertia=[0 0 0]  ProductsOfInertiaUnits=kg*m^2  BasedOnType=DensityFromFile  Density=1000  DensityUnits=kg/m^3  DoExposeReferenceFrame=on  SerializedFrames=<Frames/>  GraphicType=FromGeometry  MarkerShape=Sphere  MarkerSize=10  GraphicVisPropType=SimpleVisualProperties  GraphicDiffuseColor=[0.5 0.5 0.5]  GraphicSpecularColor=[0.5 0.5 0.5 1.0]  GraphicAmbientColor=[0.15 0.15 0.15 1.0]  GraphicEmissiveColor=[0.0 0.0 0.0 1.0]  GraphicShininess=75  GraphicOpacity=1.0
  Reference Frame : sm_lib/Frames and Transforms/Reference Frame
  Rigid Transform6 : sm_lib/Frames and Transforms/Rigid Transform  TranslationMethod=Cartesian  TranslationStandardOffset=0  TranslationStandardOffsetUnits=m  TranslationStandardAxis=+Z  TranslationCartesianOffset=[0 -0.06 0]  TranslationCartesianOffsetUnits=m  TranslationROffset=0  TranslationROffsetUnits=m  TranslationZOffset=0  TranslationZOffsetUnits=m  TranslationThetaOffset=0  TranslationThetaOffsetUnits=deg  RotationMethod=RotationMatrix  RotationAngleUnits=deg  RotationStandardAxis=+Z  RotationAngle=0.0  RotationArbitraryAxis=[0 0 1]  FollAlignAxisA=+X  BaseAlignAxisA=+Y  FollAlignAxisB=+Y  BaseAlignAxisB=+Z  RotationSequenceAxes=FollowerAxes  RotationSequence=XYX  RotationSequenceAngles=[0 0 0]  RotationSequenceAnglesUnits=deg  RotationMatrix="[0 -1 0;  0 0 -1; 1 0 0]"  Quaternion=[1 0 0 0]
  F : PMIOPort  Side=Right
  F1 : PMIOPort  Port=2  Side=Left
  connections:
  Rigid Transform6/RConn1 -- F/RConn1
  File Solid2/RConn1 -- F1/RConn1 -- Reference Frame/RConn1 -- Rigid Transform6/LConn1

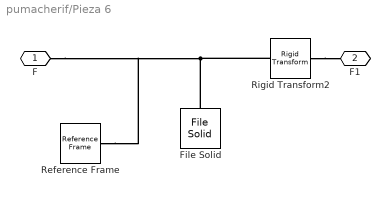
== system pumacherif/Pieza 6 ==
  File Solid : sm_lib/Body Elements/File Solid  ExtGeomFileName=C:\Users\enzoc\Desktop\TP PUMA\puma\Pieza 6_Predeterminado_sldprt.STL  UnitType=Custom  ExtGeomFileUnits=in  StepReaderType=HEX  ExportConvexHullGeometry=off  InertiaType=Custom  Mass=1  MassUnits=kg  CenterOfMass=[0 0 0]  CenterOfMassUnits=m  MomentsOfInertia=[1 1 1]  MomentsOfInertiaUnits=kg*m^2  ProductsOfInertia=[0 0 0]  ProductsOfInertiaUnits=kg*m^2  BasedOnType=DensityFromFile  Density=1000  DensityUnits=kg/m^3  DoExposeReferenceFrame=on  SerializedFrames=<Frames/>  GraphicType=FromGeometry  MarkerShape=Sphere  MarkerSize=10  GraphicVisPropType=SimpleVisualProperties  GraphicDiffuseColor=[0.5 0.5 0.5]  GraphicSpecularColor=[0.5 0.5 0.5 1.0]  GraphicAmbientColor=[0.15 0.15 0.15 1.0]  GraphicEmissiveColor=[0.0 0.0 0.0 1.0]  GraphicShininess=75  GraphicOpacity=1.0
  Reference Frame : sm_lib/Frames and Transforms/Reference Frame
  Rigid Transform2 : sm_lib/Frames and Transforms/Rigid Transform  TranslationMethod=None  TranslationStandardOffset=0  TranslationStandardOffsetUnits=m  TranslationStandardAxis=+Z  TranslationCartesianOffset=[0 0 0]  TranslationCartesianOffsetUnits=m  TranslationROffset=0  TranslationROffsetUnits=m  TranslationZOffset=0  TranslationZOffsetUnits=m  TranslationThetaOffset=0  TranslationThetaOffsetUnits=deg  RotationMethod=None  RotationAngleUnits=deg  RotationStandardAxis=+Z  RotationAngle=0.0  RotationArbitraryAxis=[0 0 1]  FollAlignAxisA=+X  BaseAlignAxisA=+Y  FollAlignAxisB=+Y  BaseAlignAxisB=+Z  RotationSequenceAxes=FollowerAxes  RotationSequence=XYX  RotationSequenceAngles=[0 0 0]  RotationSequenceAnglesUnits=deg  RotationMatrix=[1 0 0; 0 1 0; 0 0 1]  Quaternion=[1 0 0 0]
  F : PMIOPort  Side=Left
  F1 : PMIOPort  Port=2  Side=Right
  connections:
  Rigid Transform2/LConn1 -- Reference Frame/RConn1 -- F/RConn1 -- File Solid/RConn1
  Rigid Transform2/RConn1 -- F1/RConn1

== matlab function pumacherif/MATLAB Function ==
  data: u input; y output
function y = jacob_inv(u)
%#eml
q1=u(1);
q2=u(2);
q3=u(3);
q=q1+q2+q3;% raccourcis de la somme des 3 angles.

d1=0.142 ;d3=0.432 ;d56=0.360 ; d4=0.038
dx=u(4);
dy=u(5);
dtheta=u(6);

c1 = cos(q1); c2 = cos(q2); c3 = cos(q3);
s1 = sin(q1); s2 = sin(q2); s3 = sin(q3);
 
jacob = [
    -d1*s1 + d3*c2*c1 + d4*s2*s1 + d56*c3*s2*c1 - d56*s3*c2*c1, -d3*s2*s1 + d56*c3*c2*s1 + d56*s3*s2*s1, -d56*c3*c2*s1 - d56*s3*s2*s1;
    d1*c1 + d3*c2*c1 - d4*s2*c1 + d56*c3*s2*s1 - d56*s3*c2*s1, d3*s2*c1 - d56*c3*c2*c1 - d56*s3*s2*c1, d56*c3*c2*c1 + d56*s3*s2*c1;
    0, -d3*c2 - d56*c3*s2 + d56*s3*c2, d56*c3*s2 - d56*s3*c2
];
y = (inv(jacob))*[ dx ; dy ; dtheta ];
